simulink model "TP5_Effets_during_entry_avec_BPs_StateFlow"  (R2022b)
settings: Solver=VariableStepAuto  StartTime=0.0  StopTime=inf  RelTol=1e-3
libraries: spsSawtoothGeneratorLib x1
settings Model: Creator=HP  LastModifiedBy=HP

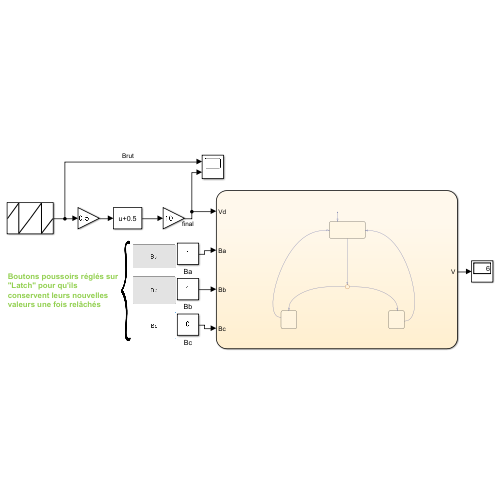
[thumbnail: Simulink's stored preview of the top-level diagram]
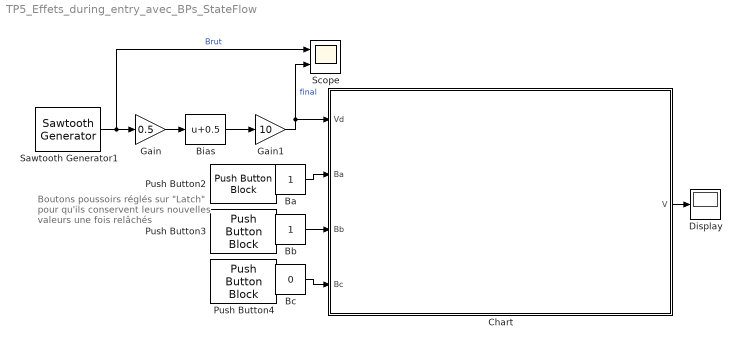
== system TP5_Effets_during_entry_avec_BPs_StateFlow ==
  note: Boutons poussoirs réglés sur
      | "Latch" pour qu'ils
      | conservent leurs nouvelles
      | valeurs une fois relâchés
  Ba : Constant
  Bb : Constant
  Bc : Constant  Value=0
  Bias : Bias  Bias=0.5  SaturateOnIntegerOverflow=off
  Chart : Stateflow chart  TreatAsAtomicUnit=on
  Display : Display
  Gain : Gain  Gain=0.5
  Gain1 : Gain  Gain=10
  Push Button2 : PushButtonBlock  ButtonText=Ba  ButtonType=Latch  OffValue=0.000000
  Push Button3 : PushButtonBlock  ButtonText=Bb  ButtonType=Latch  OffValue=0.000000
  Push Button4 : PushButtonBlock  ButtonText=Bc  ButtonType=Latch  OffValue=0.000000
  Sawtooth Generator1 : spsSawtoothGeneratorLib/Sawtooth Generator  Freq=0.5  Phase=180  Ts=0
  Scope : Scope  NumInputPorts=2
  wires:
  Gain/1 -> Bias/1
  Bias/1 -> Gain1/1
  Chart/1(V) -> Display/1
  Gain1/1 -> Scope/2, Chart/1(Vd)  "final"
  Ba/1 -> Chart/2(Ba)
  Bb/1 -> Chart/3(Bb)
  Bc/1 -> Chart/4(Bc)
  Sawtooth Generator1/1 -> Scope/1, Gain/1  "Brut"

== stateflow chart TP5_Effets_during_entry_avec_BPs_StateFlow/Chart ==
  state repos
    entry:
    V = 0;
  state variable
    during:
    V = Vd;
  state Fixe
    entry:
    V = Vd;
  (default) -> repos
  variable -> repos : [Ba == 0 || Bb == 0 && Bc == 0]
  Fixe -> repos : [Ba == 0 || Bb == 0 && Bc == 0]
  repos -> (junction 6) : [Ba == 1]
  (junction 6) -> variable [order 1] : [Bb ==  0 && Bc == 1]
  (junction 6) -> Fixe [order 2] : [Bb == 1 && Bc == 0]
  data: Vd input; Ba input; V output; Bb input; Bc input
